simulink model "dcdc1"  (R2026a)
settings: Solver=ode23t  StopTime=0.2  MaxStep=1/20e6  EnableMultiTasking=on
undefined symbols (not defined in the file): C, C0, Diode_class, f, IdealSwitch_class, L, L0, PWMGenerator_DC_DC__class, R, Vin
libraries: fl_lib x16, nesl_utility x7, simulink_need_slupdate x2, eeGeneralControl x1, eePwmGenerator x1
settings Model: Creator=almazaya  LastModifiedBy=mads
settings SolverCC: ZeroCrossAlgorithm=Non-adaptive
settings DataIOCC: SignalLoggingSaveFormat=ModelDataLogs
settings OptimizationCC: InitFltsAndDblsToZero=on
settings DebuggingCC: SaveWithParameterizedLinksMsg=none  UnderspecifiedInitializationDetection=Classic
settings HardwareCC: ProdHWDeviceType=32-bit Generic
settings GRTTargetCC: CombineOutputUpdateFcns=off  GRTInterface=on
settings SimscapeCC: SimscapeLogType=none  SimscapeLogDataHistory=5000.0

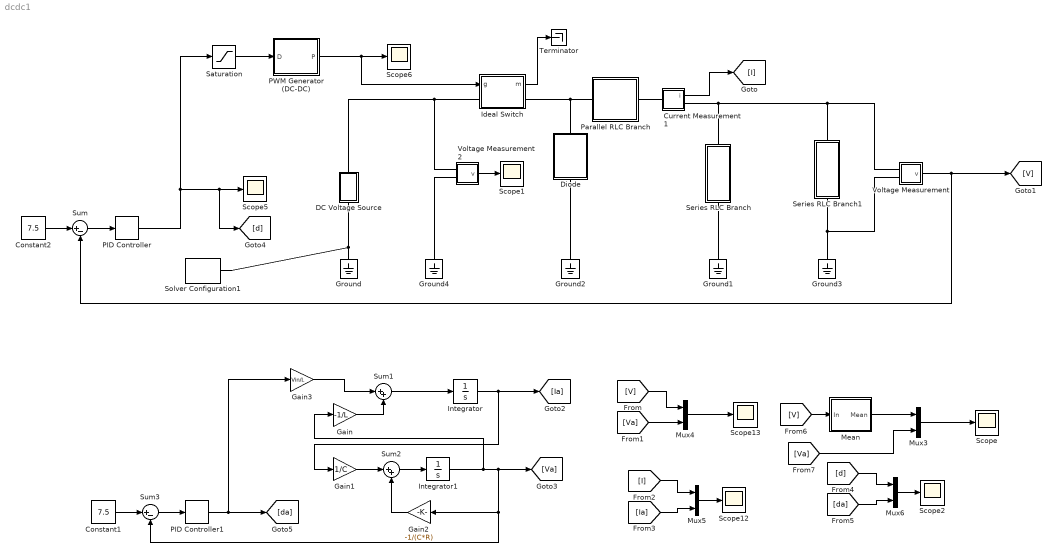
== system dcdc1 ==
  Constant1 : Constant  Value=7.5
  Constant2 : Constant  Value=7.5
  Current Measurement1 : Subsystem
      settings: OpenFcn=elec.conv.unmask(gcb);
  DC Voltage Source : Subsystem
      settings: OpenFcn=elec.conv.unmask(gcb);
  Diode : Subsystem
      settings: OpenFcn=elec.conv.unmask(gcb);
  Gain : Gain  Gain=-1/L
  Gain1 : Gain  Gain=1/C
  Gain2 : Gain  Gain=-1/(C*R)
  Gain3 : Gain  Gain=Vin/L
  Ground{,1..4} (5 alike) : fl_lib/Electrical/Electrical Elements/Electrical Reference
  Ideal Switch : Subsystem
      settings: OpenFcn=elec.conv.unmask(gcb);
  Integrator : Integrator  InitialCondition=L0
  Integrator1 : Integrator  InitialCondition=C0
  Mean : Subsystem
      settings: OpenFcn=elec.conv.unmask(gcb);
  Mux{3..6} (4 alike) : Mux  Inputs=2
  PID Controller : simulink_need_slupdate/PID Controller  P=1  I=10  D=0
  PID Controller1 : simulink_need_slupdate/PID Controller  P=1  I=10  D=0
  PWM Generator (DC-DC) : Subsystem
      settings: OpenFcn=elec.conv.unmask(gcb);
  Parallel RLC Branch : Subsystem
      settings: AttributesFormatString=\n  OpenFcn=elec.conv.unmask(gcb);
  Saturation : Saturate  UpperLimit=1  LowerLimit=0
  Scope{,1..2,5..6,12..13} (7 alike) : Scope
      Scope settings: ActiveDisplayYMinimum=6.36616  ActiveDisplayYMaximum=7.63353  DataLoggingMaxPoints=5000000
      Scope1 settings: ActiveDisplayYMinimum=9.5  ActiveDisplayYMaximum=10.5
      Scope12 settings: ActiveDisplayYMinimum=0.86155  ActiveDisplayYMaximum=1.22883  DataLoggingMaxPoints=500000000
      Scope13 settings: ActiveDisplayYMinimum=6.39728  ActiveDisplayYMaximum=7.62252  DataLoggingMaxPoints=500000000  DataLoggingVariableName=ScopeData2
      Scope2 settings: ActiveDisplayYMinimum=0.50904  ActiveDisplayYMaximum=0.54416  DataLoggingMaxPoints=500000000  DataLoggingVariableName=ScopeData3
      Scope5 settings: ActiveDisplayYMinimum=-164.33889  ActiveDisplayYMaximum=129.37099  DataLoggingMaxPoints=5000000  DataLoggingVariableName=ScopeData5
      Scope6 settings: ActiveDisplayYMinimum=-0.125  ActiveDisplayYMaximum=1.125  DataLoggingMaxPoints=5000000  DataLoggingVariableName=ScopeData6
  Series RLC Branch : Subsystem
      settings: OpenFcn=elec.conv.unmask(gcb);
  Series RLC Branch1 : Subsystem
      settings: OpenFcn=elec.conv.unmask(gcb);
  Solver Configuration1 : nesl_utility/Solver Configuration  PhysicalDomain=network_engine_domain  SubClassName=solver  LeftPortType=input  RightPortType=generic  Tones=[]  Harmonics=[]  SimulateNoise=off  Profile=off  UseLocalSampling=off  EnableSwitchedLinearOptims=on  FrequencyDomain=off  UseCCode=off  RelTol=0.001  AbsTol=0.001  MinStep=1e-09  ToWorkspace=off  RevertToSquareIcSolve=off  NumHomotopyIterations=100  PhasorMode=off  PhasorModeNumHarmonics=1  ConsistencySolver=NEWTON_XTOL_AFTER_FTOL  CanonicalOrdering=CANONICAL  OptimizeIntermediates=OPTIMIZED  IndexReductionMethod=DerivativeReplacement  DoDC=off  ResidualTolerance=1e-09  ConsistencyTolSource=GLOBAL  ConsistencyAbsTol=0.001  ConsistencyRelTol=0.001  ConsistencyTolFactor=0.001  UseLocalSolver=off  LocalSolverChoice=NE_BACKWARD_EULER_ADVANCER  ResolveIndetEquations=on  FunctionEvalNumThread=1  LocalSolverSampleTime=0.001  DoFixedCost=off  MaxNonlinIter=3  MaxModeIter=2  ComputeImpulses=off  ImpulseIterations=2  LinearAlgebra=auto  LinearAlgebraNumThread=0  EquationFormulation=NE_TIME_EF  DelaysMemoryBudget=1024  AutomaticFiltering=on  FilteringTimeConstant=0.001  PartitionStorageMethod=AS_NEEDED  PartitionMemoryBudget=1024  PartitionMethod=ROBUST  MultibodyUseLocalSolver=off  MultibodyLocalSolverChoice=ODE1  MultibodyLocalSolverSampleTime=0.001
  Sum : Sum  Inputs=|+-
  Sum1 : Sum  Inputs=|++
  Sum2 : Sum  Inputs=|++
  Sum3 : Sum  Inputs=|+-
  Terminator : Terminator
  Voltage Measurement : Subsystem
      settings: OpenFcn=elec.conv.unmask(gcb);
  Voltage Measurement2 : Subsystem
      settings: OpenFcn=elec.conv.unmask(gcb);
  wires:
  Ideal Switch/1(m) -> Terminator/1
  Voltage Measurement/1(v) -> [V], Sum/2
  Voltage Measurement2/1(v) -> Scope1/1
  Constant2/1 -> Sum/1
  PID Controller/1 -> [d], Scope5/1, Saturation/1
  Sum/1 -> PID Controller/1
  Saturation/1 -> PWM Generator (DC-DC)/1(D)
  PWM Generator (DC-DC)/1(P) -> Ideal Switch/1(g), Scope6/1
  Sum1/1 -> Integrator/1
  Gain/1 -> Sum1/2
  Integrator/1 -> [Ia], Gain1/1
  Gain1/1 -> Sum2/1
  Sum2/1 -> Integrator1/1
  Gain2/1 -> Sum2/2
  Constant1/1 -> Sum3/1
  Sum3/1 -> PID Controller1/1
  Gain3/1 -> Sum1/1
  PID Controller1/1 -> Gain3/1, [da]
  Integrator1/1 -> Gain/1, [Va], Gain2/1, Sum3/2
  Mean/1(Mean) -> Mux3/1
  Mux5/1 -> Scope12/1
  [V] -> Mux4/1
  [I] -> Mux5/1
  [Va] -> Mux4/2
  Mux4/1 -> Scope13/1
  [Ia] -> Mux5/2
  Current Measurement1/1(i) -> [I]
  Mux3/1 -> Scope/1
  [da] -> Mux6/2
  [d] -> Mux6/1
  Mux6/1 -> Scope2/1
  [V] -> Mean/1(In)
  [Va] -> Mux3/2
  connections:
  Voltage Measurement/LConn2 -- Ground3/LConn1 -- Series RLC Branch1/RConn1
  Current Measurement1/RConn1 -- Voltage Measurement/LConn1 -- Series RLC Branch1/LConn1 -- Series RLC Branch/LConn1
  Diode/RConn1 -- Parallel RLC Branch/LConn1 -- Ideal Switch/RConn1
  DC Voltage Source/LConn1 -- Ground/LConn1 -- Solver Configuration1/RConn1
  Ideal Switch/LConn1 -- DC Voltage Source/RConn1 -- Voltage Measurement2/LConn1
  Ground4/LConn1 -- Voltage Measurement2/LConn2
  Parallel RLC Branch/RConn1 -- Current Measurement1/LConn1
  Ground2/LConn1 -- Diode/LConn1
  Series RLC Branch/RConn1 -- Ground1/LConn1

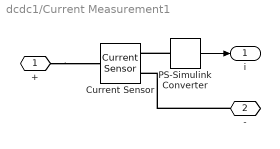
== system dcdc1/Current Measurement1 ==
  Current Sensor : fl_lib/Electrical/Electrical Sensors/Current Sensor
  PS-Simulink Converter : nesl_utility/PS-Simulink Converter  PhysicalDomain=network_engine_domain  SubClassName=ps_output  LeftPortType=input  RightPortType=output  PseudoPeriodic=off  Frequencies=[]  VectorFormat=1-D array  Unit=A  AffineConversion=off
  + : PMIOPort  Side=Left
  - : PMIOPort  Port=2  Side=Right
  i : Outport  VectorParamsAs1DForOutWhenUnconnected=off
  wires:
  PS-Simulink Converter/1 -> i/1
  connections:
  +/RConn1 -- Current Sensor/LConn1
  -/RConn1 -- Current Sensor/RConn2
  PS-Simulink Converter/LConn1 -- Current Sensor/RConn1

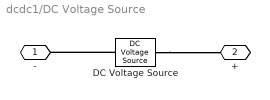
== system dcdc1/DC Voltage Source ==
  DC Voltage Source : fl_lib/Electrical/Electrical Sources/DC Voltage Source  v0=Vin V
  - : PMIOPort  Side=Left
  + : PMIOPort  Port=2  Side=Right
  connections:
  DC Voltage Source/RConn1 -- -/RConn1
  DC Voltage Source/LConn1 -- +/RConn1

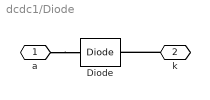
== system dcdc1/Diode ==
  Diode : fl_lib/Electrical/Electrical Elements/Diode  Vf=Diode_class(1e-06,Inf,0,0).objParamMappingDerived.NewDerivedParam.Vf V  Ron=Diode_class(1e-06,Inf,0,0).objParamMappingDerived.NewDerivedParam.Ron Ohm  Goff=Diode_class(1e-06,Inf,0,0).objParamMappingDerived.NewDerivedParam.Goff 1/Ohm  i_specify=off  i_priority=None  i=0 A  i_nominal_specify=off  i_nominal_value=1  i_nominal_unit=A  v_specify=off  v_priority=None  v=0 V  v_nominal_specify=off  v_nominal_value=1  v_nominal_unit=V
  a : PMIOPort  Side=Left
  k : PMIOPort  Port=2  Side=Right
  connections:
  k/RConn1 -- Diode/RConn1
  a/RConn1 -- Diode/LConn1

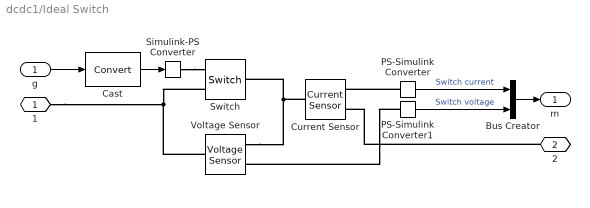
== system dcdc1/Ideal Switch ==
  g : Inport
  Bus Creator : BusCreator  Inputs=2
  Cast : DataTypeConversion  SaturateOnIntegerOverflow=off  RndMeth=Floor
  Current Sensor : fl_lib/Electrical/Electrical Sensors/Current Sensor
  PS-Simulink Converter : nesl_utility/PS-Simulink Converter  PhysicalDomain=network_engine_domain  SubClassName=ps_output  LeftPortType=input  RightPortType=output  PseudoPeriodic=off  Frequencies=[]  VectorFormat=1-D array  Unit=1  AffineConversion=off
  PS-Simulink Converter1 : nesl_utility/PS-Simulink Converter  PhysicalDomain=network_engine_domain  SubClassName=ps_output  LeftPortType=input  RightPortType=output  PseudoPeriodic=off  Frequencies=[]  VectorFormat=1-D array  Unit=1  AffineConversion=off
  Simulink-PS Converter : nesl_utility/Simulink-PS Converter  PhysicalDomain=network_engine_domain  SubClassName=ps_input  LeftPortType=input  RightPortType=output  PseudoPeriodic=off  Frequencies=[]  NoiseDistribution=none  NoiseParameters=[]  Unit=1  AffineConversion=off  FilteringAndDerivatives=provide  SimscapeFilterOrder=1  InputFilterTimeConstant=0.001  UdotUserProvided=0
  Switch : fl_lib/Electrical/Electrical Elements/Switch  R_closed=IdealSwitch_class(0.001,100000,Inf).objParamMappingDerived.NewDerivedParam.R_closed Ohm  G_open=IdealSwitch_class(0.001,100000,Inf).objParamMappingDerived.NewDerivedParam.G_open 1/Ohm  Threshold=0.5  i_specify=off  i_priority=None  i=0 A  i_nominal_specify=off  i_nominal_value=1  i_nominal_unit=A  v_specify=off  v_priority=None  v=0 V  v_nominal_specify=off  v_nominal_value=1  v_nominal_unit=V
  Voltage Sensor : fl_lib/Electrical/Electrical Sensors/Voltage Sensor
  1 : PMIOPort  Side=Left
  2 : PMIOPort  Port=2  Side=Right
  m : Outport  VectorParamsAs1DForOutWhenUnconnected=off
  wires:
  Cast/1 -> Simulink-PS Converter/1
  PS-Simulink Converter/1 -> Bus Creator/1  "Switch current"
  Bus Creator/1 -> m/1
  g/1 -> Cast/1
  PS-Simulink Converter1/1 -> Bus Creator/2  "Switch voltage"
  connections:
  Current Sensor/LConn1 -- Voltage Sensor/RConn2 -- Switch/LConn1
  1/RConn1 -- Voltage Sensor/LConn1 -- Switch/RConn2
  PS-Simulink Converter1/LConn1 -- Voltage Sensor/RConn1
  PS-Simulink Converter/LConn1 -- Current Sensor/RConn1
  2/RConn1 -- Current Sensor/RConn2
  Simulink-PS Converter/RConn1 -- Switch/RConn1

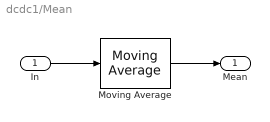
== system dcdc1/Mean ==
  In : Inport
  Moving Average : eeGeneralControl/Moving Average  VariantControl=Variant1  LabelModeActiveChoice=Discrete  f=f  x0=7  BufferSize=8192  Ts=0
  Mean : Outport  VectorParamsAs1DForOutWhenUnconnected=off
  wires:
  Moving Average/1 -> Mean/1
  In/1 -> Moving Average/1

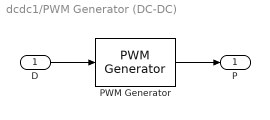
== system dcdc1/PWM Generator (DC-DC) ==
  D : Inport
  PWM Generator : eePwmGenerator/PWM Generator  CarrCount=Up  Tper=PWMGenerator_DC_DC__class(f).objParamMappingDerived.NewDerivedParam.Tper  Tdelay=0  Ts=0
  P : Outport  VectorParamsAs1DForOutWhenUnconnected=off
  wires:
  D/1 -> PWM Generator/1
  PWM Generator/1 -> P/1

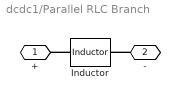
== system dcdc1/Parallel RLC Branch ==
  Inductor : fl_lib/Electrical/Electrical Elements/Inductor  l=L H  r=0 Ohm  g=1e-9 1/Ohm  i_specify=off  i_priority=None  i=0 A  i_nominal_specify=off  i_nominal_value=1  i_nominal_unit=A  v_specify=off  v_priority=None  v=0 V  v_nominal_specify=off  v_nominal_value=1  v_nominal_unit=V  i_L_specify=on  i_L_priority=High  i_L=L0 A  i_L_nominal_specify=off  i_L_nominal_value=1  i_L_nominal_unit=A
  + : PMIOPort  Side=Left
  - : PMIOPort  Port=2  Side=Right
  connections:
  -/RConn1 -- Inductor/RConn1
  Inductor/LConn1 -- +/RConn1

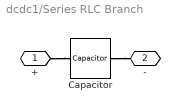
== system dcdc1/Series RLC Branch ==
  Capacitor : fl_lib/Electrical/Electrical Elements/Capacitor  c=C F  r=1e-6 Ohm  g=0 1/Ohm  i_specify=off  i_priority=None  i=0 A  i_nominal_specify=off  i_nominal_value=1  i_nominal_unit=A  v_specify=off  v_priority=None  v=0 V  v_nominal_specify=off  v_nominal_value=1  v_nominal_unit=V  vc_specify=on  vc_priority=High  vc=C0 V  vc_nominal_specify=off  vc_nominal_value=1  vc_nominal_unit=V
  + : PMIOPort  Side=Left
  - : PMIOPort  Port=2  Side=Right
  connections:
  Capacitor/RConn1 -- -/RConn1
  +/RConn1 -- Capacitor/LConn1

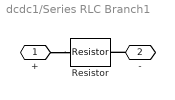
== system dcdc1/Series RLC Branch1 ==
  Resistor : fl_lib/Electrical/Electrical Elements/Resistor  R=R Ohm  i_specify=off  i_priority=None  i=0 A  i_nominal_specify=off  i_nominal_value=1  i_nominal_unit=A  v_specify=off  v_priority=None  v=0 V  v_nominal_specify=off  v_nominal_value=1  v_nominal_unit=V
  + : PMIOPort  Side=Left
  - : PMIOPort  Port=2  Side=Right
  connections:
  +/RConn1 -- Resistor/LConn1
  -/RConn1 -- Resistor/RConn1

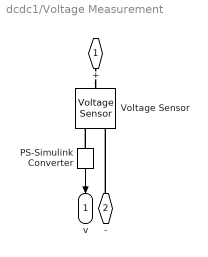
== system dcdc1/Voltage Measurement ==
  PS-Simulink Converter : nesl_utility/PS-Simulink Converter  PhysicalDomain=network_engine_domain  SubClassName=ps_output  LeftPortType=input  RightPortType=output  PseudoPeriodic=off  Frequencies=[]  VectorFormat=1-D array  Unit=V  AffineConversion=off
  Voltage Sensor : fl_lib/Electrical/Electrical Sensors/Voltage Sensor
  + : PMIOPort  Side=Left
  - : PMIOPort  Port=2  Side=Left
  v : Outport  VectorParamsAs1DForOutWhenUnconnected=off
  wires:
  PS-Simulink Converter/1 -> v/1
  connections:
  PS-Simulink Converter/LConn1 -- Voltage Sensor/RConn1
  -/RConn1 -- Voltage Sensor/RConn2
  +/RConn1 -- Voltage Sensor/LConn1

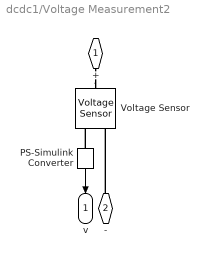
== system dcdc1/Voltage Measurement2 ==
  PS-Simulink Converter : nesl_utility/PS-Simulink Converter  PhysicalDomain=network_engine_domain  SubClassName=ps_output  LeftPortType=input  RightPortType=output  PseudoPeriodic=off  Frequencies=[]  VectorFormat=1-D array  Unit=V  AffineConversion=off
  Voltage Sensor : fl_lib/Electrical/Electrical Sensors/Voltage Sensor
  + : PMIOPort  Side=Left
  - : PMIOPort  Port=2  Side=Left
  v : Outport  VectorParamsAs1DForOutWhenUnconnected=off
  wires:
  PS-Simulink Converter/1 -> v/1
  connections:
  PS-Simulink Converter/LConn1 -- Voltage Sensor/RConn1
  -/RConn1 -- Voltage Sensor/RConn2
  +/RConn1 -- Voltage Sensor/LConn1
